simulink model "Ten_phase_nine_leg_relocated_L3_L7"  (R2025b)
settings: Solver=VariableStepAuto  StartTime=0.0  StopTime=0.05  FixedStep=1e-6  MaxStep=1e-6  RelTol=1e-4
values from neighbouring files (symbols this model uses):
  bias_current = 5    [parameters_for_AMB_topology.m]
  half_SW_Ts = SW_Ts*0.5    (= 2.5e-05)    [parameters_for_AMB_topology.m]
  K_i = 2*pi*f_c*R_value/U_dc    (= 47.1238898038)    [parameters_for_AMB_topology.m]
  K_p = 2*pi*f_c*L_value/U_dc    (= 0.0235619449019)    [parameters_for_AMB_topology.m]
  R_value = 1    [parameters_for_AMB_topology.m]
  SW_Ts = 1/(SW_frequency)    (= 5e-05)    [parameters_for_AMB_topology.m]
libraries: fl_lib x61, simulink x39, nesl_utility x29, eeGeneralControl x28, ee_lib x19
(part 4 of 4)

== system Ten_phase_nine_leg_relocated_L3_L7/PWM_gen5 ==
  U : Inport
  Gain : Gain  Gain=15  OutDataTypeStr=double
  Gain1 : Gain  Gain=15  OutDataTypeStr=double
  NOT : Logic  Operator=NOT  IconShape=distinctive  AllPortsSameDT=off  OutDataTypeStr=boolean
  On-Off Delay : eeGeneralControl/On-Off Delay  LabelModeActiveChoice=Continuous  Td_on=1e-6  Td_off=0  IC=0  Ts=0
      settings: LibrarySourceBlock=ee_sl_lib/General Control/On-Off Delay
  On-Off Delay1 : eeGeneralControl/On-Off Delay  LabelModeActiveChoice=Continuous  Td_on=1e-6  Td_off=0  IC=0  Ts=0
      settings: LibrarySourceBlock=ee_sl_lib/General Control/On-Off Delay
  Relational Operator2 : RelationalOperator  OutDataTypeStr=boolean  RndMeth=Simplest  InputSameDT=off
  Repeating Sequence : simulink/Sources/Repeating Sequence  rep_seq_t=[0 half_SW_Ts SW_Ts]  rep_seq_y=[0 1 0]
  PWMH : Outport
  PWML : Outport  Port=2
  wires:
  Repeating Sequence/1 -> Relational Operator2/2
  U/1 -> Relational Operator2/1
  Relational Operator2/1 -> NOT/1, On-Off Delay1/1
  NOT/1 -> On-Off Delay/1
  On-Off Delay1/1 -> Gain/1
  Gain/1 -> PWMH/1
  On-Off Delay/1 -> Gain1/1
  Gain1/1 -> PWML/1

== system Ten_phase_nine_leg_relocated_L3_L7/PWM_gen6 ==
  U : Inport
  Gain : Gain  Gain=15  OutDataTypeStr=double
  Gain1 : Gain  Gain=15  OutDataTypeStr=double
  NOT : Logic  Operator=NOT  IconShape=distinctive  AllPortsSameDT=off  OutDataTypeStr=boolean
  On-Off Delay : eeGeneralControl/On-Off Delay  LabelModeActiveChoice=Continuous  Td_on=1e-6  Td_off=0  IC=0  Ts=0
      settings: LibrarySourceBlock=ee_sl_lib/General Control/On-Off Delay
  On-Off Delay1 : eeGeneralControl/On-Off Delay  LabelModeActiveChoice=Continuous  Td_on=1e-6  Td_off=0  IC=0  Ts=0
      settings: LibrarySourceBlock=ee_sl_lib/General Control/On-Off Delay
  Relational Operator2 : RelationalOperator  OutDataTypeStr=boolean  RndMeth=Simplest  InputSameDT=off
  Repeating Sequence : simulink/Sources/Repeating Sequence  rep_seq_t=[0 half_SW_Ts SW_Ts]  rep_seq_y=[0 1 0]
  PWMH : Outport
  PWML : Outport  Port=2
  wires:
  Repeating Sequence/1 -> Relational Operator2/2
  U/1 -> Relational Operator2/1
  Relational Operator2/1 -> NOT/1, On-Off Delay1/1
  NOT/1 -> On-Off Delay/1
  On-Off Delay1/1 -> Gain/1
  Gain/1 -> PWMH/1
  On-Off Delay/1 -> Gain1/1
  Gain1/1 -> PWML/1

== system Ten_phase_nine_leg_relocated_L3_L7/PWM_gen7 ==
  U : Inport
  Gain : Gain  Gain=15  OutDataTypeStr=double
  Gain1 : Gain  Gain=15  OutDataTypeStr=double
  NOT : Logic  Operator=NOT  IconShape=distinctive  AllPortsSameDT=off  OutDataTypeStr=boolean
  On-Off Delay : eeGeneralControl/On-Off Delay  LabelModeActiveChoice=Continuous  Td_on=1e-6  Td_off=0  IC=0  Ts=0
      settings: LibrarySourceBlock=ee_sl_lib/General Control/On-Off Delay
  On-Off Delay1 : eeGeneralControl/On-Off Delay  LabelModeActiveChoice=Continuous  Td_on=1e-6  Td_off=0  IC=0  Ts=0
      settings: LibrarySourceBlock=ee_sl_lib/General Control/On-Off Delay
  Relational Operator2 : RelationalOperator  OutDataTypeStr=boolean  RndMeth=Simplest  InputSameDT=off
  Repeating Sequence : simulink/Sources/Repeating Sequence  rep_seq_t=[0 half_SW_Ts SW_Ts]  rep_seq_y=[0 1 0]
  PWMH : Outport
  PWML : Outport  Port=2
  wires:
  Repeating Sequence/1 -> Relational Operator2/2
  U/1 -> Relational Operator2/1
  Relational Operator2/1 -> NOT/1, On-Off Delay1/1
  NOT/1 -> On-Off Delay/1
  On-Off Delay1/1 -> Gain/1
  Gain/1 -> PWMH/1
  On-Off Delay/1 -> Gain1/1
  Gain1/1 -> PWML/1

== system Ten_phase_nine_leg_relocated_L3_L7/PWM_gen8 ==
  U : Inport
  Gain : Gain  Gain=15  OutDataTypeStr=double
  Gain1 : Gain  Gain=15  OutDataTypeStr=double
  NOT : Logic  Operator=NOT  IconShape=distinctive  AllPortsSameDT=off  OutDataTypeStr=boolean
  On-Off Delay : eeGeneralControl/On-Off Delay  LabelModeActiveChoice=Continuous  Td_on=1e-6  Td_off=0  IC=0  Ts=0
      settings: LibrarySourceBlock=ee_sl_lib/General Control/On-Off Delay
  On-Off Delay1 : eeGeneralControl/On-Off Delay  LabelModeActiveChoice=Continuous  Td_on=1e-6  Td_off=0  IC=0  Ts=0
      settings: LibrarySourceBlock=ee_sl_lib/General Control/On-Off Delay
  Relational Operator2 : RelationalOperator  OutDataTypeStr=boolean  RndMeth=Simplest  InputSameDT=off
  Repeating Sequence : simulink/Sources/Repeating Sequence  rep_seq_t=[0 half_SW_Ts SW_Ts]  rep_seq_y=[0 1 0]
  PWMH : Outport
  PWML : Outport  Port=2
  wires:
  Repeating Sequence/1 -> Relational Operator2/2
  U/1 -> Relational Operator2/1
  Relational Operator2/1 -> NOT/1, On-Off Delay1/1
  NOT/1 -> On-Off Delay/1
  On-Off Delay1/1 -> Gain/1
  Gain/1 -> PWMH/1
  On-Off Delay/1 -> Gain1/1
  Gain1/1 -> PWML/1

== system Ten_phase_nine_leg_relocated_L3_L7/RL_load ==
  Current Sensor2 : fl_lib/Electrical/Electrical Sensors/Current Sensor
  Inductor2 : fl_lib/Electrical/Electrical Elements/Inductor  l=L_value H  r=0 Ohm  g=1e-9 1/Ohm  i_specify=off  i_priority=None  i=0 A  i_nominal_specify=off  i_nominal_value=1  i_nominal_unit=A  v_specify=off  v_priority=None  v=0 V  v_nominal_specify=off  v_nominal_value=1  v_nominal_unit=V  i_L_specify=off  i_L_priority=High  i_L=0 A  i_L_nominal_specify=off  i_L_nominal_value=1  i_L_nominal_unit=A
  PS-Simulink Converter : nesl_utility/PS-Simulink Converter  PhysicalDomain=network_engine_domain  SubClassName=ps_output  LeftPortType=input  RightPortType=output  PseudoPeriodic=off  Frequencies=[]  VectorFormat=inherit  Unit=inherit  AffineConversion=off
  Resistor2 : fl_lib/Electrical/Electrical Elements/Resistor  R=R_value Ohm  i_specify=off  i_priority=None  i=0 A  i_nominal_specify=off  i_nominal_value=1  i_nominal_unit=A  v_specify=off  v_priority=None  v=0 V  v_nominal_specify=off  v_nominal_value=1  v_nominal_unit=V
  L : PMIOPort  Side=Left
  R : PMIOPort  Port=2  Side=Right
  i_fbk : Outport
  wires:
  PS-Simulink Converter/1 -> i_fbk/1
  connections:
  Inductor2/LConn1 -- Resistor2/RConn1
  Resistor2/LConn1 -- L/RConn1
  Current Sensor2/LConn1 -- Inductor2/RConn1
  Current Sensor2/RConn2 -- R/RConn1
  PS-Simulink Converter/LConn1 -- Current Sensor2/RConn1

== system Ten_phase_nine_leg_relocated_L3_L7/RL_load1 ==
  Current Sensor2 : fl_lib/Electrical/Electrical Sensors/Current Sensor
  Inductor2 : fl_lib/Electrical/Electrical Elements/Inductor  l=L_value H  r=0 Ohm  g=1e-9 1/Ohm  i_specify=off  i_priority=None  i=0 A  i_nominal_specify=off  i_nominal_value=1  i_nominal_unit=A  v_specify=off  v_priority=None  v=0 V  v_nominal_specify=off  v_nominal_value=1  v_nominal_unit=V  i_L_specify=off  i_L_priority=High  i_L=0 A  i_L_nominal_specify=off  i_L_nominal_value=1  i_L_nominal_unit=A
  PS-Simulink Converter : nesl_utility/PS-Simulink Converter  PhysicalDomain=network_engine_domain  SubClassName=ps_output  LeftPortType=input  RightPortType=output  PseudoPeriodic=off  Frequencies=[]  VectorFormat=inherit  Unit=inherit  AffineConversion=off
  Resistor2 : fl_lib/Electrical/Electrical Elements/Resistor  R=R_value Ohm  i_specify=off  i_priority=None  i=0 A  i_nominal_specify=off  i_nominal_value=1  i_nominal_unit=A  v_specify=off  v_priority=None  v=0 V  v_nominal_specify=off  v_nominal_value=1  v_nominal_unit=V
  L : PMIOPort  Side=Left
  R : PMIOPort  Port=2  Side=Right
  i_fbk : Outport
  wires:
  PS-Simulink Converter/1 -> i_fbk/1
  connections:
  Inductor2/LConn1 -- Resistor2/RConn1
  Resistor2/LConn1 -- L/RConn1
  Current Sensor2/LConn1 -- Inductor2/RConn1
  Current Sensor2/RConn2 -- R/RConn1
  PS-Simulink Converter/LConn1 -- Current Sensor2/RConn1

== system Ten_phase_nine_leg_relocated_L3_L7/RL_load2 ==
  Current Sensor2 : fl_lib/Electrical/Electrical Sensors/Current Sensor
  Inductor2 : fl_lib/Electrical/Electrical Elements/Inductor  l=L_value H  r=0 Ohm  g=1e-9 1/Ohm  i_specify=off  i_priority=None  i=0 A  i_nominal_specify=off  i_nominal_value=1  i_nominal_unit=A  v_specify=off  v_priority=None  v=0 V  v_nominal_specify=off  v_nominal_value=1  v_nominal_unit=V  i_L_specify=off  i_L_priority=High  i_L=0 A  i_L_nominal_specify=off  i_L_nominal_value=1  i_L_nominal_unit=A
  PS-Simulink Converter : nesl_utility/PS-Simulink Converter  PhysicalDomain=network_engine_domain  SubClassName=ps_output  LeftPortType=input  RightPortType=output  PseudoPeriodic=off  Frequencies=[]  VectorFormat=inherit  Unit=inherit  AffineConversion=off
  Resistor2 : fl_lib/Electrical/Electrical Elements/Resistor  R=R_value Ohm  i_specify=off  i_priority=None  i=0 A  i_nominal_specify=off  i_nominal_value=1  i_nominal_unit=A  v_specify=off  v_priority=None  v=0 V  v_nominal_specify=off  v_nominal_value=1  v_nominal_unit=V
  L : PMIOPort  Side=Left
  R : PMIOPort  Port=2  Side=Right
  i_fbk : Outport
  wires:
  PS-Simulink Converter/1 -> i_fbk/1
  connections:
  Inductor2/LConn1 -- Resistor2/RConn1
  Resistor2/LConn1 -- L/RConn1
  Current Sensor2/LConn1 -- Inductor2/RConn1
  Current Sensor2/RConn2 -- R/RConn1
  PS-Simulink Converter/LConn1 -- Current Sensor2/RConn1

== system Ten_phase_nine_leg_relocated_L3_L7/RL_load3 ==
  Current Sensor2 : fl_lib/Electrical/Electrical Sensors/Current Sensor
  Inductor2 : fl_lib/Electrical/Electrical Elements/Inductor  l=L_value H  r=0 Ohm  g=1e-9 1/Ohm  i_specify=off  i_priority=None  i=0 A  i_nominal_specify=off  i_nominal_value=1  i_nominal_unit=A  v_specify=off  v_priority=None  v=0 V  v_nominal_specify=off  v_nominal_value=1  v_nominal_unit=V  i_L_specify=off  i_L_priority=High  i_L=0 A  i_L_nominal_specify=off  i_L_nominal_value=1  i_L_nominal_unit=A
  PS-Simulink Converter : nesl_utility/PS-Simulink Converter  PhysicalDomain=network_engine_domain  SubClassName=ps_output  LeftPortType=input  RightPortType=output  PseudoPeriodic=off  Frequencies=[]  VectorFormat=inherit  Unit=inherit  AffineConversion=off
  Resistor2 : fl_lib/Electrical/Electrical Elements/Resistor  R=R_value Ohm  i_specify=off  i_priority=None  i=0 A  i_nominal_specify=off  i_nominal_value=1  i_nominal_unit=A  v_specify=off  v_priority=None  v=0 V  v_nominal_specify=off  v_nominal_value=1  v_nominal_unit=V
  L : PMIOPort  Side=Left
  R : PMIOPort  Port=2  Side=Right
  i_fbk : Outport
  wires:
  PS-Simulink Converter/1 -> i_fbk/1
  connections:
  Inductor2/LConn1 -- Resistor2/RConn1
  Resistor2/LConn1 -- L/RConn1
  Current Sensor2/LConn1 -- Inductor2/RConn1
  Current Sensor2/RConn2 -- R/RConn1
  PS-Simulink Converter/LConn1 -- Current Sensor2/RConn1

== system Ten_phase_nine_leg_relocated_L3_L7/RL_load4 ==
  Current Sensor2 : fl_lib/Electrical/Electrical Sensors/Current Sensor
  Inductor2 : fl_lib/Electrical/Electrical Elements/Inductor  l=L_value H  r=0 Ohm  g=1e-9 1/Ohm  i_specify=off  i_priority=None  i=0 A  i_nominal_specify=off  i_nominal_value=1  i_nominal_unit=A  v_specify=off  v_priority=None  v=0 V  v_nominal_specify=off  v_nominal_value=1  v_nominal_unit=V  i_L_specify=off  i_L_priority=High  i_L=0 A  i_L_nominal_specify=off  i_L_nominal_value=1  i_L_nominal_unit=A
  PS-Simulink Converter : nesl_utility/PS-Simulink Converter  PhysicalDomain=network_engine_domain  SubClassName=ps_output  LeftPortType=input  RightPortType=output  PseudoPeriodic=off  Frequencies=[]  VectorFormat=inherit  Unit=inherit  AffineConversion=off
  Resistor2 : fl_lib/Electrical/Electrical Elements/Resistor  R=R_value Ohm  i_specify=off  i_priority=None  i=0 A  i_nominal_specify=off  i_nominal_value=1  i_nominal_unit=A  v_specify=off  v_priority=None  v=0 V  v_nominal_specify=off  v_nominal_value=1  v_nominal_unit=V
  L : PMIOPort  Side=Left
  R : PMIOPort  Port=2  Side=Right
  i_fbk : Outport
  wires:
  PS-Simulink Converter/1 -> i_fbk/1
  connections:
  Inductor2/LConn1 -- Resistor2/RConn1
  Resistor2/LConn1 -- L/RConn1
  Current Sensor2/LConn1 -- Inductor2/RConn1
  Current Sensor2/RConn2 -- R/RConn1
  PS-Simulink Converter/LConn1 -- Current Sensor2/RConn1

== system Ten_phase_nine_leg_relocated_L3_L7/RL_load5 ==
  Current Sensor2 : fl_lib/Electrical/Electrical Sensors/Current Sensor
  Inductor2 : fl_lib/Electrical/Electrical Elements/Inductor  l=L_value H  r=0 Ohm  g=1e-9 1/Ohm  i_specify=off  i_priority=None  i=0 A  i_nominal_specify=off  i_nominal_value=1  i_nominal_unit=A  v_specify=off  v_priority=None  v=0 V  v_nominal_specify=off  v_nominal_value=1  v_nominal_unit=V  i_L_specify=off  i_L_priority=High  i_L=0 A  i_L_nominal_specify=off  i_L_nominal_value=1  i_L_nominal_unit=A
  PS-Simulink Converter : nesl_utility/PS-Simulink Converter  PhysicalDomain=network_engine_domain  SubClassName=ps_output  LeftPortType=input  RightPortType=output  PseudoPeriodic=off  Frequencies=[]  VectorFormat=inherit  Unit=inherit  AffineConversion=off
  Resistor2 : fl_lib/Electrical/Electrical Elements/Resistor  R=R_value Ohm  i_specify=off  i_priority=None  i=0 A  i_nominal_specify=off  i_nominal_value=1  i_nominal_unit=A  v_specify=off  v_priority=None  v=0 V  v_nominal_specify=off  v_nominal_value=1  v_nominal_unit=V
  L : PMIOPort  Side=Left
  R : PMIOPort  Port=2  Side=Right
  i_fbk : Outport
  wires:
  PS-Simulink Converter/1 -> i_fbk/1
  connections:
  Inductor2/LConn1 -- Resistor2/RConn1
  Resistor2/LConn1 -- L/RConn1
  Current Sensor2/LConn1 -- Inductor2/RConn1
  Current Sensor2/RConn2 -- R/RConn1
  PS-Simulink Converter/LConn1 -- Current Sensor2/RConn1

== system Ten_phase_nine_leg_relocated_L3_L7/RL_load6 ==
  Current Sensor2 : fl_lib/Electrical/Electrical Sensors/Current Sensor
  Inductor2 : fl_lib/Electrical/Electrical Elements/Inductor  l=L_value H  r=0 Ohm  g=1e-9 1/Ohm  i_specify=off  i_priority=None  i=0 A  i_nominal_specify=off  i_nominal_value=1  i_nominal_unit=A  v_specify=off  v_priority=None  v=0 V  v_nominal_specify=off  v_nominal_value=1  v_nominal_unit=V  i_L_specify=off  i_L_priority=High  i_L=0 A  i_L_nominal_specify=off  i_L_nominal_value=1  i_L_nominal_unit=A
  PS-Simulink Converter : nesl_utility/PS-Simulink Converter  PhysicalDomain=network_engine_domain  SubClassName=ps_output  LeftPortType=input  RightPortType=output  PseudoPeriodic=off  Frequencies=[]  VectorFormat=inherit  Unit=inherit  AffineConversion=off
  Resistor2 : fl_lib/Electrical/Electrical Elements/Resistor  R=R_value Ohm  i_specify=off  i_priority=None  i=0 A  i_nominal_specify=off  i_nominal_value=1  i_nominal_unit=A  v_specify=off  v_priority=None  v=0 V  v_nominal_specify=off  v_nominal_value=1  v_nominal_unit=V
  L : PMIOPort  Side=Left
  R : PMIOPort  Port=2  Side=Right
  i_fbk : Outport
  wires:
  PS-Simulink Converter/1 -> i_fbk/1
  connections:
  Inductor2/LConn1 -- Resistor2/RConn1
  Resistor2/LConn1 -- L/RConn1
  Current Sensor2/LConn1 -- Inductor2/RConn1
  Current Sensor2/RConn2 -- R/RConn1
  PS-Simulink Converter/LConn1 -- Current Sensor2/RConn1

== system Ten_phase_nine_leg_relocated_L3_L7/RL_load7 ==
  Current Sensor2 : fl_lib/Electrical/Electrical Sensors/Current Sensor
  Inductor2 : fl_lib/Electrical/Electrical Elements/Inductor  l=L_value H  r=0 Ohm  g=1e-9 1/Ohm  i_specify=off  i_priority=None  i=0 A  i_nominal_specify=off  i_nominal_value=1  i_nominal_unit=A  v_specify=off  v_priority=None  v=0 V  v_nominal_specify=off  v_nominal_value=1  v_nominal_unit=V  i_L_specify=off  i_L_priority=High  i_L=0 A  i_L_nominal_specify=off  i_L_nominal_value=1  i_L_nominal_unit=A
  PS-Simulink Converter : nesl_utility/PS-Simulink Converter  PhysicalDomain=network_engine_domain  SubClassName=ps_output  LeftPortType=input  RightPortType=output  PseudoPeriodic=off  Frequencies=[]  VectorFormat=inherit  Unit=inherit  AffineConversion=off
  Resistor2 : fl_lib/Electrical/Electrical Elements/Resistor  R=R_value Ohm  i_specify=off  i_priority=None  i=0 A  i_nominal_specify=off  i_nominal_value=1  i_nominal_unit=A  v_specify=off  v_priority=None  v=0 V  v_nominal_specify=off  v_nominal_value=1  v_nominal_unit=V
  L : PMIOPort  Side=Left
  R : PMIOPort  Port=2  Side=Right
  i_fbk : Outport
  wires:
  PS-Simulink Converter/1 -> i_fbk/1
  connections:
  Inductor2/LConn1 -- Resistor2/RConn1
  Resistor2/LConn1 -- L/RConn1
  Current Sensor2/LConn1 -- Inductor2/RConn1
  Current Sensor2/RConn2 -- R/RConn1
  PS-Simulink Converter/LConn1 -- Current Sensor2/RConn1

== system Ten_phase_nine_leg_relocated_L3_L7/RL_load8 ==
  Current Sensor2 : fl_lib/Electrical/Electrical Sensors/Current Sensor
  Inductor2 : fl_lib/Electrical/Electrical Elements/Inductor  l=L_value H  r=0 Ohm  g=1e-9 1/Ohm  i_specify=off  i_priority=None  i=0 A  i_nominal_specify=off  i_nominal_value=1  i_nominal_unit=A  v_specify=off  v_priority=None  v=0 V  v_nominal_specify=off  v_nominal_value=1  v_nominal_unit=V  i_L_specify=off  i_L_priority=High  i_L=0 A  i_L_nominal_specify=off  i_L_nominal_value=1  i_L_nominal_unit=A
  PS-Simulink Converter : nesl_utility/PS-Simulink Converter  PhysicalDomain=network_engine_domain  SubClassName=ps_output  LeftPortType=input  RightPortType=output  PseudoPeriodic=off  Frequencies=[]  VectorFormat=inherit  Unit=inherit  AffineConversion=off
  Resistor2 : fl_lib/Electrical/Electrical Elements/Resistor  R=R_value Ohm  i_specify=off  i_priority=None  i=0 A  i_nominal_specify=off  i_nominal_value=1  i_nominal_unit=A  v_specify=off  v_priority=None  v=0 V  v_nominal_specify=off  v_nominal_value=1  v_nominal_unit=V
  L : PMIOPort  Side=Left
  R : PMIOPort  Port=2  Side=Right
  i_fbk : Outport
  wires:
  PS-Simulink Converter/1 -> i_fbk/1
  connections:
  Inductor2/LConn1 -- Resistor2/RConn1
  Resistor2/LConn1 -- L/RConn1
  Current Sensor2/LConn1 -- Inductor2/RConn1
  Current Sensor2/RConn2 -- R/RConn1
  PS-Simulink Converter/LConn1 -- Current Sensor2/RConn1

== system Ten_phase_nine_leg_relocated_L3_L7/RL_load9 ==
  Current Sensor2 : fl_lib/Electrical/Electrical Sensors/Current Sensor
  Inductor2 : fl_lib/Electrical/Electrical Elements/Inductor  l=L_value H  r=0 Ohm  g=1e-9 1/Ohm  i_specify=off  i_priority=None  i=0 A  i_nominal_specify=off  i_nominal_value=1  i_nominal_unit=A  v_specify=off  v_priority=None  v=0 V  v_nominal_specify=off  v_nominal_value=1  v_nominal_unit=V  i_L_specify=off  i_L_priority=High  i_L=0 A  i_L_nominal_specify=off  i_L_nominal_value=1  i_L_nominal_unit=A
  PS-Simulink Converter : nesl_utility/PS-Simulink Converter  PhysicalDomain=network_engine_domain  SubClassName=ps_output  LeftPortType=input  RightPortType=output  PseudoPeriodic=off  Frequencies=[]  VectorFormat=inherit  Unit=inherit  AffineConversion=off
  Resistor2 : fl_lib/Electrical/Electrical Elements/Resistor  R=R_value Ohm  i_specify=off  i_priority=None  i=0 A  i_nominal_specify=off  i_nominal_value=1  i_nominal_unit=A  v_specify=off  v_priority=None  v=0 V  v_nominal_specify=off  v_nominal_value=1  v_nominal_unit=V
  L : PMIOPort  Side=Left
  R : PMIOPort  Port=2  Side=Right
  i_fbk : Outport
  wires:
  PS-Simulink Converter/1 -> i_fbk/1
  connections:
  Inductor2/LConn1 -- Resistor2/RConn1
  Resistor2/LConn1 -- L/RConn1
  Current Sensor2/LConn1 -- Inductor2/RConn1
  Current Sensor2/RConn2 -- R/RConn1
  PS-Simulink Converter/LConn1 -- Current Sensor2/RConn1

== system Ten_phase_nine_leg_relocated_L3_L7/ref_delay ==
  ref1 : Inport
  ref2 : Inport  Port=2
  ctrl : Inport  Port=3
  Constant8 : Constant  Value=0
  Switch : Switch  Criteria=u2 > Threshold  SaturateOnIntegerOverflow=off  InputSameDT=off
  Switch1 : Switch  Criteria=u2 > Threshold  SaturateOnIntegerOverflow=off  InputSameDT=off
  delay1 : Outport
  delay2 : Outport  Port=2
  wires:
  Switch1/1 -> delay2/1
  Constant8/1 -> Switch/3, Switch1/3
  ref2/1 -> Switch1/1
  Switch/1 -> delay1/1
  ref1/1 -> Switch/1
  ctrl/1 -> Switch1/2, Switch/2

== system Ten_phase_nine_leg_relocated_L3_L7/ref_delay1 ==
  ref1 : Inport
  ref2 : Inport  Port=2
  ctrl : Inport  Port=3
  Constant8 : Constant  Value=0
  Switch : Switch  Criteria=u2 > Threshold  SaturateOnIntegerOverflow=off  InputSameDT=off
  Switch1 : Switch  Criteria=u2 > Threshold  SaturateOnIntegerOverflow=off  InputSameDT=off
  delay1 : Outport
  delay2 : Outport  Port=2
  wires:
  Switch1/1 -> delay2/1
  Constant8/1 -> Switch/3, Switch1/3
  ref2/1 -> Switch1/1
  Switch/1 -> delay1/1
  ref1/1 -> Switch/1
  ctrl/1 -> Switch1/2, Switch/2

== system Ten_phase_nine_leg_relocated_L3_L7/ref_delay2 ==
  ref1 : Inport
  ref2 : Inport  Port=2
  ctrl : Inport  Port=3
  Constant8 : Constant  Value=0
  Switch : Switch  Criteria=u2 > Threshold  SaturateOnIntegerOverflow=off  InputSameDT=off
  Switch1 : Switch  Criteria=u2 > Threshold  SaturateOnIntegerOverflow=off  InputSameDT=off
  delay1 : Outport
  delay2 : Outport  Port=2
  wires:
  Switch1/1 -> delay2/1
  Constant8/1 -> Switch/3, Switch1/3
  ref2/1 -> Switch1/1
  Switch/1 -> delay1/1
  ref1/1 -> Switch/1
  ctrl/1 -> Switch1/2, Switch/2

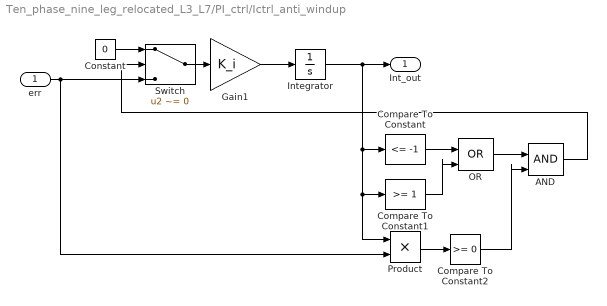
== system Ten_phase_nine_leg_relocated_L3_L7/PI_ctrl/Ictrl_anti_windup ==
  err : Inport
  AND : Logic  IconShape=distinctive  AllPortsSameDT=off  OutDataTypeStr=boolean
  Compare To Constant : simulink/Logic and Bit Operations/Compare To Constant  relop=<=  const=-1  OutDataTypeStr=boolean
  Compare To Constant1 : simulink/Logic and Bit Operations/Compare To Constant  relop=>=  const=1  OutDataTypeStr=boolean
  Compare To Constant2 : simulink/Logic and Bit Operations/Compare To Constant  relop=>=  const=0  OutDataTypeStr=boolean
  Constant : Constant  Value=0
  Gain1 : Gain  Gain=K_i
  Integrator : Integrator  LimitOutput=on  UpperSaturationLimit=1  LowerSaturationLimit=-1
  OR : Logic  Operator=OR  IconShape=distinctive  AllPortsSameDT=off  OutDataTypeStr=boolean
  Product : Product
  Switch : Switch  Criteria=u2 ~= 0  SaturateOnIntegerOverflow=off  InputSameDT=off
  Int_out : Outport
  wires:
  Compare To Constant2/1 -> AND/2
  Product/1 -> Compare To Constant2/1
  AND/1 -> Switch/2
  Constant/1 -> Switch/1
  Compare To Constant1/1 -> OR/2
  Switch/1 -> Gain1/1
  Gain1/1 -> Integrator/1
  Integrator/1 -> Int_out/1, Product/1, Compare To Constant1/1, Compare To Constant/1
  OR/1 -> AND/1
  Compare To Constant/1 -> OR/1
  err/1 -> Product/2, Switch/3

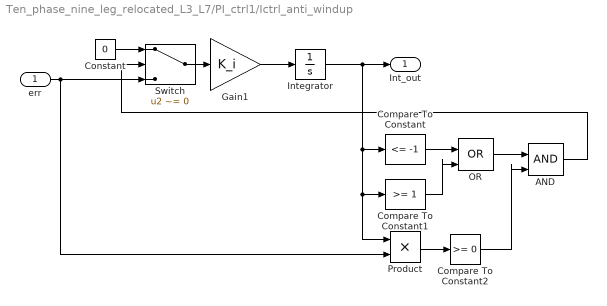
== system Ten_phase_nine_leg_relocated_L3_L7/PI_ctrl1/Ictrl_anti_windup ==
  err : Inport
  AND : Logic  IconShape=distinctive  AllPortsSameDT=off  OutDataTypeStr=boolean
  Compare To Constant : simulink/Logic and Bit Operations/Compare To Constant  relop=<=  const=-1  OutDataTypeStr=boolean
  Compare To Constant1 : simulink/Logic and Bit Operations/Compare To Constant  relop=>=  const=1  OutDataTypeStr=boolean
  Compare To Constant2 : simulink/Logic and Bit Operations/Compare To Constant  relop=>=  const=0  OutDataTypeStr=boolean
  Constant : Constant  Value=0
  Gain1 : Gain  Gain=K_i
  Integrator : Integrator  LimitOutput=on  UpperSaturationLimit=1  LowerSaturationLimit=-1
  OR : Logic  Operator=OR  IconShape=distinctive  AllPortsSameDT=off  OutDataTypeStr=boolean
  Product : Product
  Switch : Switch  Criteria=u2 ~= 0  SaturateOnIntegerOverflow=off  InputSameDT=off
  Int_out : Outport
  wires:
  Compare To Constant2/1 -> AND/2
  Product/1 -> Compare To Constant2/1
  AND/1 -> Switch/2
  Constant/1 -> Switch/1
  Compare To Constant1/1 -> OR/2
  Switch/1 -> Gain1/1
  Gain1/1 -> Integrator/1
  Integrator/1 -> Int_out/1, Product/1, Compare To Constant1/1, Compare To Constant/1
  OR/1 -> AND/1
  Compare To Constant/1 -> OR/1
  err/1 -> Product/2, Switch/3

== system Ten_phase_nine_leg_relocated_L3_L7/PI_ctrl2/Ictrl_anti_windup ==
  err : Inport
  AND : Logic  IconShape=distinctive  AllPortsSameDT=off  OutDataTypeStr=boolean
  Compare To Constant : simulink/Logic and Bit Operations/Compare To Constant  relop=<=  const=-1  OutDataTypeStr=boolean
  Compare To Constant1 : simulink/Logic and Bit Operations/Compare To Constant  relop=>=  const=1  OutDataTypeStr=boolean
  Compare To Constant2 : simulink/Logic and Bit Operations/Compare To Constant  relop=>=  const=0  OutDataTypeStr=boolean
  Constant : Constant  Value=0
  Gain1 : Gain  Gain=K_i
  Integrator : Integrator  LimitOutput=on  UpperSaturationLimit=1  LowerSaturationLimit=-1
  OR : Logic  Operator=OR  IconShape=distinctive  AllPortsSameDT=off  OutDataTypeStr=boolean
  Product : Product
  Switch : Switch  Criteria=u2 ~= 0  SaturateOnIntegerOverflow=off  InputSameDT=off
  Int_out : Outport
  wires:
  Compare To Constant2/1 -> AND/2
  Product/1 -> Compare To Constant2/1
  AND/1 -> Switch/2
  Constant/1 -> Switch/1
  Compare To Constant1/1 -> OR/2
  Switch/1 -> Gain1/1
  Gain1/1 -> Integrator/1
  Integrator/1 -> Int_out/1, Product/1, Compare To Constant1/1, Compare To Constant/1
  OR/1 -> AND/1
  Compare To Constant/1 -> OR/1
  err/1 -> Product/2, Switch/3

== system Ten_phase_nine_leg_relocated_L3_L7/PI_ctrl3/Ictrl_anti_windup ==
  err : Inport
  AND : Logic  IconShape=distinctive  AllPortsSameDT=off  OutDataTypeStr=boolean
  Compare To Constant : simulink/Logic and Bit Operations/Compare To Constant  relop=<=  const=-1  OutDataTypeStr=boolean
  Compare To Constant1 : simulink/Logic and Bit Operations/Compare To Constant  relop=>=  const=1  OutDataTypeStr=boolean
  Compare To Constant2 : simulink/Logic and Bit Operations/Compare To Constant  relop=>=  const=0  OutDataTypeStr=boolean
  Constant : Constant  Value=0
  Gain1 : Gain  Gain=K_i
  Integrator : Integrator  LimitOutput=on  UpperSaturationLimit=1  LowerSaturationLimit=-1
  OR : Logic  Operator=OR  IconShape=distinctive  AllPortsSameDT=off  OutDataTypeStr=boolean
  Product : Product
  Switch : Switch  Criteria=u2 ~= 0  SaturateOnIntegerOverflow=off  InputSameDT=off
  Int_out : Outport
  wires:
  Compare To Constant2/1 -> AND/2
  Product/1 -> Compare To Constant2/1
  AND/1 -> Switch/2
  Constant/1 -> Switch/1
  Compare To Constant1/1 -> OR/2
  Switch/1 -> Gain1/1
  Gain1/1 -> Integrator/1
  Integrator/1 -> Int_out/1, Product/1, Compare To Constant1/1, Compare To Constant/1
  OR/1 -> AND/1
  Compare To Constant/1 -> OR/1
  err/1 -> Product/2, Switch/3

== system Ten_phase_nine_leg_relocated_L3_L7/PI_ctrl4/Ictrl_anti_windup ==
  err : Inport
  AND : Logic  IconShape=distinctive  AllPortsSameDT=off  OutDataTypeStr=boolean
  Compare To Constant : simulink/Logic and Bit Operations/Compare To Constant  relop=<=  const=-1  OutDataTypeStr=boolean
  Compare To Constant1 : simulink/Logic and Bit Operations/Compare To Constant  relop=>=  const=1  OutDataTypeStr=boolean
  Compare To Constant2 : simulink/Logic and Bit Operations/Compare To Constant  relop=>=  const=0  OutDataTypeStr=boolean
  Constant : Constant  Value=0
  Gain1 : Gain  Gain=K_i
  Integrator : Integrator  LimitOutput=on  UpperSaturationLimit=1  LowerSaturationLimit=-1
  OR : Logic  Operator=OR  IconShape=distinctive  AllPortsSameDT=off  OutDataTypeStr=boolean
  Product : Product
  Switch : Switch  Criteria=u2 ~= 0  SaturateOnIntegerOverflow=off  InputSameDT=off
  Int_out : Outport
  wires:
  Compare To Constant2/1 -> AND/2
  Product/1 -> Compare To Constant2/1
  AND/1 -> Switch/2
  Constant/1 -> Switch/1
  Compare To Constant1/1 -> OR/2
  Switch/1 -> Gain1/1
  Gain1/1 -> Integrator/1
  Integrator/1 -> Int_out/1, Product/1, Compare To Constant1/1, Compare To Constant/1
  OR/1 -> AND/1
  Compare To Constant/1 -> OR/1
  err/1 -> Product/2, Switch/3

== system Ten_phase_nine_leg_relocated_L3_L7/PI_ctrl5/Ictrl_anti_windup ==
  err : Inport
  AND : Logic  IconShape=distinctive  AllPortsSameDT=off  OutDataTypeStr=boolean
  Compare To Constant : simulink/Logic and Bit Operations/Compare To Constant  relop=<=  const=-1  OutDataTypeStr=boolean
  Compare To Constant1 : simulink/Logic and Bit Operations/Compare To Constant  relop=>=  const=1  OutDataTypeStr=boolean
  Compare To Constant2 : simulink/Logic and Bit Operations/Compare To Constant  relop=>=  const=0  OutDataTypeStr=boolean
  Constant : Constant  Value=0
  Gain1 : Gain  Gain=K_i
  Integrator : Integrator  LimitOutput=on  UpperSaturationLimit=1  LowerSaturationLimit=-1
  OR : Logic  Operator=OR  IconShape=distinctive  AllPortsSameDT=off  OutDataTypeStr=boolean
  Product : Product
  Switch : Switch  Criteria=u2 ~= 0  SaturateOnIntegerOverflow=off  InputSameDT=off
  Int_out : Outport
  wires:
  Compare To Constant2/1 -> AND/2
  Product/1 -> Compare To Constant2/1
  AND/1 -> Switch/2
  Constant/1 -> Switch/1
  Compare To Constant1/1 -> OR/2
  Switch/1 -> Gain1/1
  Gain1/1 -> Integrator/1
  Integrator/1 -> Int_out/1, Product/1, Compare To Constant1/1, Compare To Constant/1
  OR/1 -> AND/1
  Compare To Constant/1 -> OR/1
  err/1 -> Product/2, Switch/3

== system Ten_phase_nine_leg_relocated_L3_L7/PI_ctrl6/Ictrl_anti_windup ==
  err : Inport
  AND : Logic  IconShape=distinctive  AllPortsSameDT=off  OutDataTypeStr=boolean
  Compare To Constant : simulink/Logic and Bit Operations/Compare To Constant  relop=<=  const=-1  OutDataTypeStr=boolean
  Compare To Constant1 : simulink/Logic and Bit Operations/Compare To Constant  relop=>=  const=1  OutDataTypeStr=boolean
  Compare To Constant2 : simulink/Logic and Bit Operations/Compare To Constant  relop=>=  const=0  OutDataTypeStr=boolean
  Constant : Constant  Value=0
  Gain1 : Gain  Gain=K_i
  Integrator : Integrator  LimitOutput=on  UpperSaturationLimit=1  LowerSaturationLimit=-1
  OR : Logic  Operator=OR  IconShape=distinctive  AllPortsSameDT=off  OutDataTypeStr=boolean
  Product : Product
  Switch : Switch  Criteria=u2 ~= 0  SaturateOnIntegerOverflow=off  InputSameDT=off
  Int_out : Outport
  wires:
  Compare To Constant2/1 -> AND/2
  Product/1 -> Compare To Constant2/1
  AND/1 -> Switch/2
  Constant/1 -> Switch/1
  Compare To Constant1/1 -> OR/2
  Switch/1 -> Gain1/1
  Gain1/1 -> Integrator/1
  Integrator/1 -> Int_out/1, Product/1, Compare To Constant1/1, Compare To Constant/1
  OR/1 -> AND/1
  Compare To Constant/1 -> OR/1
  err/1 -> Product/2, Switch/3

== system Ten_phase_nine_leg_relocated_L3_L7/PI_ctrl7/Ictrl_anti_windup ==
  err : Inport
  AND : Logic  IconShape=distinctive  AllPortsSameDT=off  OutDataTypeStr=boolean
  Compare To Constant : simulink/Logic and Bit Operations/Compare To Constant  relop=<=  const=-1  OutDataTypeStr=boolean
  Compare To Constant1 : simulink/Logic and Bit Operations/Compare To Constant  relop=>=  const=1  OutDataTypeStr=boolean
  Compare To Constant2 : simulink/Logic and Bit Operations/Compare To Constant  relop=>=  const=0  OutDataTypeStr=boolean
  Constant : Constant  Value=0
  Gain1 : Gain  Gain=K_i
  Integrator : Integrator  LimitOutput=on  UpperSaturationLimit=1  LowerSaturationLimit=-1
  OR : Logic  Operator=OR  IconShape=distinctive  AllPortsSameDT=off  OutDataTypeStr=boolean
  Product : Product
  Switch : Switch  Criteria=u2 ~= 0  SaturateOnIntegerOverflow=off  InputSameDT=off
  Int_out : Outport
  wires:
  Compare To Constant2/1 -> AND/2
  Product/1 -> Compare To Constant2/1
  AND/1 -> Switch/2
  Constant/1 -> Switch/1
  Compare To Constant1/1 -> OR/2
  Switch/1 -> Gain1/1
  Gain1/1 -> Integrator/1
  Integrator/1 -> Int_out/1, Product/1, Compare To Constant1/1, Compare To Constant/1
  OR/1 -> AND/1
  Compare To Constant/1 -> OR/1
  err/1 -> Product/2, Switch/3

== system Ten_phase_nine_leg_relocated_L3_L7/PI_ctrl8/Ictrl_anti_windup ==
  err : Inport
  AND : Logic  IconShape=distinctive  AllPortsSameDT=off  OutDataTypeStr=boolean
  Compare To Constant : simulink/Logic and Bit Operations/Compare To Constant  relop=<=  const=-1  OutDataTypeStr=boolean
  Compare To Constant1 : simulink/Logic and Bit Operations/Compare To Constant  relop=>=  const=1  OutDataTypeStr=boolean
  Compare To Constant2 : simulink/Logic and Bit Operations/Compare To Constant  relop=>=  const=0  OutDataTypeStr=boolean
  Constant : Constant  Value=0
  Gain1 : Gain  Gain=K_i
  Integrator : Integrator  LimitOutput=on  UpperSaturationLimit=1  LowerSaturationLimit=-1
  OR : Logic  Operator=OR  IconShape=distinctive  AllPortsSameDT=off  OutDataTypeStr=boolean
  Product : Product
  Switch : Switch  Criteria=u2 ~= 0  SaturateOnIntegerOverflow=off  InputSameDT=off
  Int_out : Outport
  wires:
  Compare To Constant2/1 -> AND/2
  Product/1 -> Compare To Constant2/1
  AND/1 -> Switch/2
  Constant/1 -> Switch/1
  Compare To Constant1/1 -> OR/2
  Switch/1 -> Gain1/1
  Gain1/1 -> Integrator/1
  Integrator/1 -> Int_out/1, Product/1, Compare To Constant1/1, Compare To Constant/1
  OR/1 -> AND/1
  Compare To Constant/1 -> OR/1
  err/1 -> Product/2, Switch/3

== system Ten_phase_nine_leg_relocated_L3_L7/PI_ctrl9/Ictrl_anti_windup ==
  err : Inport
  AND : Logic  IconShape=distinctive  AllPortsSameDT=off  OutDataTypeStr=boolean
  Compare To Constant : simulink/Logic and Bit Operations/Compare To Constant  relop=<=  const=-1  OutDataTypeStr=boolean
  Compare To Constant1 : simulink/Logic and Bit Operations/Compare To Constant  relop=>=  const=1  OutDataTypeStr=boolean
  Compare To Constant2 : simulink/Logic and Bit Operations/Compare To Constant  relop=>=  const=0  OutDataTypeStr=boolean
  Constant : Constant  Value=0
  Gain1 : Gain  Gain=K_i
  Integrator : Integrator  LimitOutput=on  UpperSaturationLimit=1  LowerSaturationLimit=-1
  OR : Logic  Operator=OR  IconShape=distinctive  AllPortsSameDT=off  OutDataTypeStr=boolean
  Product : Product
  Switch : Switch  Criteria=u2 ~= 0  SaturateOnIntegerOverflow=off  InputSameDT=off
  Int_out : Outport
  wires:
  Compare To Constant2/1 -> AND/2
  Product/1 -> Compare To Constant2/1
  AND/1 -> Switch/2
  Constant/1 -> Switch/1
  Compare To Constant1/1 -> OR/2
  Switch/1 -> Gain1/1
  Gain1/1 -> Integrator/1
  Integrator/1 -> Int_out/1, Product/1, Compare To Constant1/1, Compare To Constant/1
  OR/1 -> AND/1
  Compare To Constant/1 -> OR/1
  err/1 -> Product/2, Switch/3

== matlab function Ten_phase_nine_leg_relocated_L3_L7/winding_voltage_to_bridge ==
  data: uw1 input; ubridge output; uw2 input; uw3 input; uw4 input; uw5 input; uw6 input; uw7 input; uw8 input; uw9 input; uw10 input
function ubridge = u_w2b(uw1, uw2, uw3, uw4, uw5, uw6, uw7, uw8, uw9, uw10)

ubridge = [0 0 0 0 0 0 0 0 0];

ubridge(5) = 0;

ubridge(3) = ubridge(5) + uw5;
ubridge(7) = ubridge(5) - uw6;

ubridge(1) = ubridge(3) + uw3 + uw1;
ubridge(2) = ubridge(3) + uw3 + uw2;
ubridge(4) = ubridge(3) + uw3 - uw4;

ubridge(6) = ubridge(7) - uw8 + uw7;
ubridge(8) = ubridge(7) - uw8 - uw9;
ubridge(9) = ubridge(7) - uw8 - uw10;

end

== matlab function Ten_phase_nine_leg_relocated_L3_L7/MATLAB Function ==
  data: u input; cmin output; cmax output
function [cmin, cmax] = minmax(u)

c_sorted = sort(u);      % 升序
cmin = c_sorted(1);      % 首 = 最小
cmax = c_sorted(end);    % 末 = 最大



end
